simulink model "Validation_Observer"  (R2025b)
settings: Solver=ode15s  StartTime=0.0  StopTime=6  RelTol=1e-3
undefined symbols (not defined in the file): A11, A12, A21, A22, Bd1, Bd2, Bu1, Bu2, CA_re, CAin_re, CB_re, L, QH_re, Qin_V_re, T_re, Tc_re, Tin_re
settings Model: Creator=Lenovo  LastModifiedBy=Lenovo

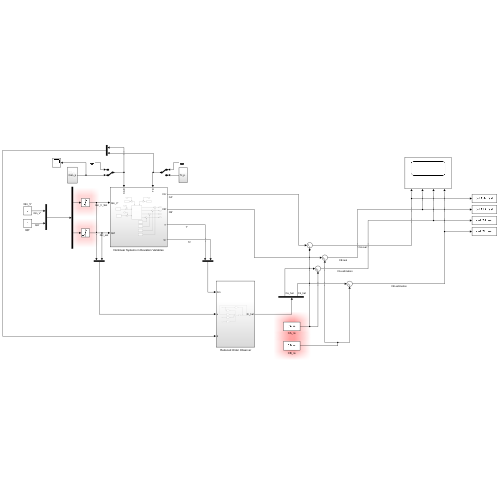
[thumbnail: Simulink's stored preview of the top-level diagram]
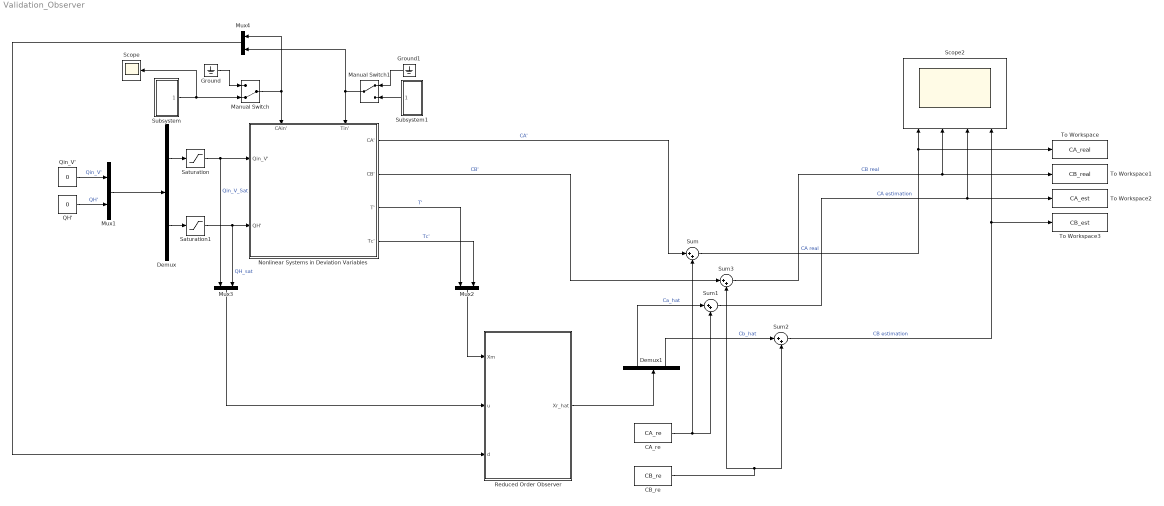
== system Validation_Observer ==
  " Reduced Order Observer" : Subsystem
  CA_re : Constant  Value=CA_re
  CB_re : Constant  Value=CB_re
  Demux : Demux  Outputs=2
  Demux1 : Demux  Outputs=2
  Ground : Ground
  Ground1 : Ground
  Manual Switch : ManualSwitch  CurrentSetting=0
  Manual Switch1 : ManualSwitch
  Mux{1..4} (4 alike) : Mux  Inputs=2
  Nonlinear Systems in Deviation Variables : Subsystem
      settings: PortSchema="{\"entries\":[{\"content\":{\"sides\":[{\"content\":{\"connectorIds\":[\"In1\",\"In2\"]},\"type\":\"ConnectorPlacement.EquallySpacedRectSide\",\"uuid\":\"3cae5363-54ae-4836-a9af-709fc6d72947\"},{\"content\":{\"connectorIds\":[\"Out1\",\"Out2\",\"Out3\",\"Out4\"],\"side\":\"RIGHT\"},\"type\":\"ConnectorPlacement.EquallySpacedRectSide\",\"uuid\":\"ac34fbf0-7c91-43b5-9805-8d79849dc8bb\"},{\"content\":{\"connectorIds\":[\"In3\",\"In4\"],\"side\":\"TOP\"},\"type\":\"ConnectorPlacement.EquallySpacedRectSide\",\"uuid\":\"0c613297-952e-4fe2-85b3-8b705fa3960d\"}]},\"type\":\"ConnectorPlacement.EquallySpacedConnector\",\"uuid\":\"6a9d9fd9-ed65-4660-8ac2-43953dadb3cb\"}],\"packageUris\":[\"http://schema.mathworks.com/mf0/Connector/R2020b\"],\"version\":\"1.0\"}"
  QH' : Constant  Value=0
  Qin_V' : Constant  Value=0
  Saturation : Saturate  UpperLimit=35-Qin_V_re  LowerLimit=5-Qin_V_re
  Saturation1 : Saturate  UpperLimit=0-QH_re  LowerLimit=-8500-QH_re
  Scope : Scope
      settings: ActiveDisplayYMinimum=-1  ActiveDisplayYMaximum=1
  Scope2 : Scope  NumInputPorts=4
      settings: ActiveDisplayYMinimum=-149.80536396754488  ActiveDisplayYMaximum=256.89603505828842  DataLoggingVariableName=ScopeData2
  Subsystem : Subsystem
  Subsystem1 : Subsystem
  Sum{,1..3} (4 alike) : Sum  Inputs=|++
  To Workspace : ToWorkspace  VariableName=CA_real  SaveFormat=Structure With Time  SampleTime=-1
  To Workspace1 : ToWorkspace  VariableName=CB_real  SaveFormat=Structure With Time  SampleTime=-1
  To Workspace2 : ToWorkspace  VariableName=CA_est  SaveFormat=Structure With Time  SampleTime=-1
  To Workspace3 : ToWorkspace  VariableName=CB_est  SaveFormat=Structure With Time  SampleTime=-1
  wires:
  Nonlinear Systems in Deviation Variables/4(Tc') -> Mux2/2  "Tc'"
  Demux/1 -> Saturation/1
  Subsystem/1(Cain_p) -> Scope/1, Manual Switch/2
  Manual Switch/1 -> Nonlinear Systems in Deviation Variables/3(CAin'), Mux4/1
  Qin_V'/1 -> Mux1/1  "Qin_V'"
  Demux/2 -> Saturation1/1
  Ground/1 -> Manual Switch/1
  Mux4/1 -> " Reduced Order Observer"/3(d)
  Mux2/1 -> " Reduced Order Observer"/1(Xm)
  Subsystem1/1(Tc_p) -> Manual Switch1/2
  Manual Switch1/1 -> Mux4/2, Nonlinear Systems in Deviation Variables/4(Tin')
  QH'/1 -> Mux1/2  "QH'"
  Nonlinear Systems in Deviation Variables/3(T') -> Mux2/1  "T'"
  Mux3/1 -> " Reduced Order Observer"/2(u)
  Saturation/1 -> Mux3/1, Nonlinear Systems in Deviation Variables/1(Qin_V')  "Qin_V_Sat"
  Saturation1/1 -> Nonlinear Systems in Deviation Variables/2(QH'), Mux3/2  "QH_sat"
  Ground1/1 -> Manual Switch1/1
  " Reduced Order Observer"/1(Xr_hat) -> Demux1/1
  Mux1/1 -> Demux/1
  Sum/1 -> To Workspace/1, Scope2/1  "CA real"
  Sum1/1 -> To Workspace2/1, Scope2/3  "CA estimation"
  Demux1/1 -> Sum1/1  "Ca_hat"
  Nonlinear Systems in Deviation Variables/1(CA') -> Sum/1  "CA'"
  CA_re/1 -> Sum1/2, Sum/2
  Sum2/1 -> To Workspace3/1, Scope2/4  "CB estimation"
  Demux1/2 -> Sum2/1  "Cb_hat"
  CB_re/1 -> Sum2/2, Sum3/2
  Sum3/1 -> To Workspace1/1, Scope2/2  "CB real"
  Nonlinear Systems in Deviation Variables/2(CB') -> Sum3/1  "CB'"

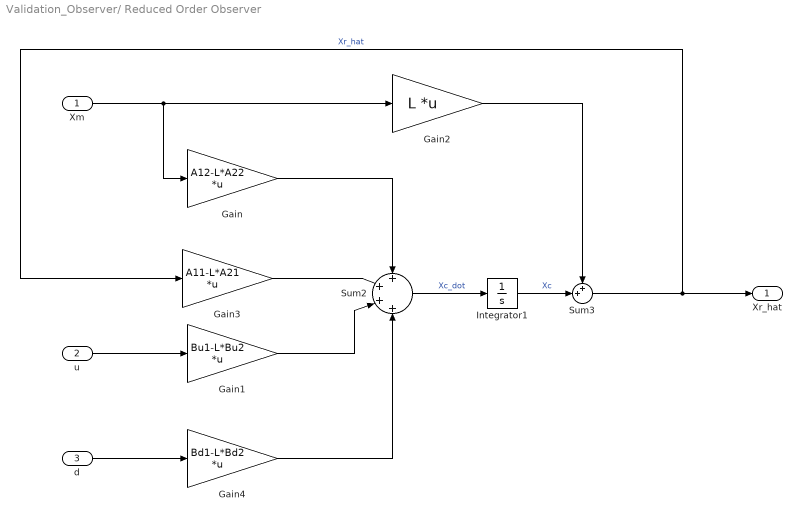
== system Validation_Observer/ Reduced Order Observer ==
  Xm : Inport
  u : Inport  Port=2
  d : Inport  Port=3
  Gain : Gain  Gain=A12-L*A22  Multiplication=Matrix(K*u)
  Gain1 : Gain  Gain=Bu1-L*Bu2  Multiplication=Matrix(K*u)
  Gain2 : Gain  Gain=L  Multiplication=Matrix(K*u)
  Gain3 : Gain  Gain=A11-L*A21  Multiplication=Matrix(K*u)
  Gain4 : Gain  Gain=Bd1-L*Bd2  Multiplication=Matrix(K*u)
  Integrator1 : Integrator
  Sum2 : Sum  Inputs=+|+|+|+
  Sum3 : Sum  Inputs=++|
  Xr_hat : Outport
  wires:
  Gain1/1 -> Sum2/3
  Sum3/1 -> Gain3/1, Xr_hat/1  "Xr_hat"
  Xm/1 -> Gain/1, Gain2/1
  Integrator1/1 -> Sum3/2  "Xc"
  Gain2/1 -> Sum3/1
  Gain/1 -> Sum2/1
  Gain3/1 -> Sum2/2
  Sum2/1 -> Integrator1/1  "Xc_dot"
  u/1 -> Gain1/1
  Gain4/1 -> Sum2/4
  d/1 -> Gain4/1

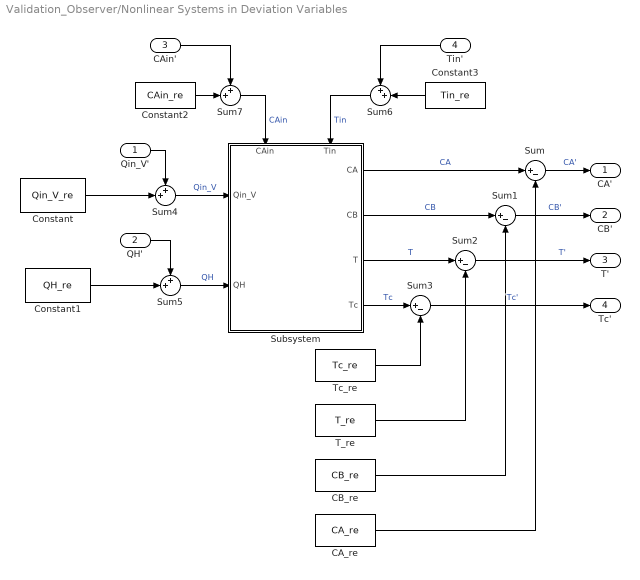
== system Validation_Observer/Nonlinear Systems in Deviation Variables ==
  Qin_V' : Inport
  QH' : Inport  Port=2
  CAin' : Inport  Port=3
  Tin' : Inport  Port=4
  CA_re : Constant  Value=CA_re
  CB_re : Constant  Value=CB_re
  Constant : Constant  Value=Qin_V_re
  Constant1 : Constant  Value=QH_re
  Constant2 : Constant  Value=CAin_re
  Constant3 : Constant  Value=Tin_re
  Subsystem : Subsystem
      settings: PortSchema="{\"entries\":[{\"content\":{\"sides\":[{\"content\":{\"connectorIds\":[\"In1\",\"In2\"]},\"type\":\"ConnectorPlacement.EquallySpacedRectSide\",\"uuid\":\"3cae5363-54ae-4836-a9af-709fc6d72947\"},{\"content\":{\"connectorIds\":[\"Out1\",\"Out2\",\"Out3\",\"Out4\"],\"side\":\"RIGHT\"},\"type\":\"ConnectorPlacement.EquallySpacedRectSide\",\"uuid\":\"ac34fbf0-7c91-43b5-9805-8d79849dc8bb\"},{\"content\":{\"connectorIds\":[\"In3\",\"In4\"],\"side\":\"TOP\"},\"type\":\"ConnectorPlacement.EquallySpacedRectSide\",\"uuid\":\"0c613297-952e-4fe2-85b3-8b705fa3960d\"}]},\"type\":\"ConnectorPlacement.EquallySpacedConnector\",\"uuid\":\"6a9d9fd9-ed65-4660-8ac2-43953dadb3cb\"}],\"packageUris\":[\"http://schema.mathworks.com/mf0/Connector/R2020b\"],\"version\":\"1.0\"}"
  Sum{,1..3} (4 alike) : Sum  Inputs=|+-
  Sum{4..7} (4 alike) : Sum  Inputs=++|
  T_re : Constant  Value=T_re
  Tc_re : Constant  Value=Tc_re
  CA' : Outport
  CB' : Outport  Port=2
  T' : Outport  Port=3
  Tc' : Outport  Port=4
  wires:
  Tc_re/1 -> Sum3/2
  Subsystem/4(Tc) -> Sum3/1  "Tc"
  Subsystem/3(T) -> Sum2/1  "T"
  Sum1/1 -> CB'/1  "CB'"
  Sum4/1 -> Subsystem/1(Qin_V)  "Qin_V"
  CB_re/1 -> Sum1/2
  Sum2/1 -> T'/1  "T'"
  Subsystem/1(CA) -> Sum/1  "CA"
  Sum/1 -> CA'/1  "CA'"
  Constant/1 -> Sum4/2
  T_re/1 -> Sum2/2
  Sum5/1 -> Subsystem/2(QH)  "QH"
  Constant1/1 -> Sum5/2
  CA_re/1 -> Sum/2
  Subsystem/2(CB) -> Sum1/1  "CB"
  QH'/1 -> Sum5/1
  Sum3/1 -> Tc'/1  "Tc'"
  Qin_V'/1 -> Sum4/1
  Constant3/1 -> Sum6/2
  Sum6/1 -> Subsystem/4(Tin)  "Tin"
  Tin'/1 -> Sum6/1
  Sum7/1 -> Subsystem/3(CAin)  "CAin"
  Constant2/1 -> Sum7/2
  CAin'/1 -> Sum7/1

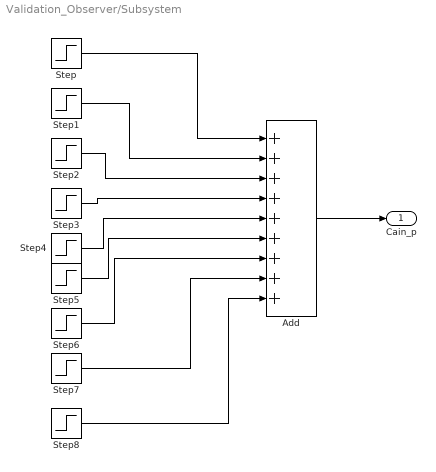
== system Validation_Observer/Subsystem ==
  Add : Sum  Inputs=+++++++++
  Step : Step  Time=0.5  After=300  SampleTime=0
  Step1 : Step  Before=300  After=150  SampleTime=0
  Step2 : Step  Time=1.5  After=-100*2  SampleTime=0
  Step3 : Step  Time=2  Before=-100*2  After=0  SampleTime=0
  Step4 : Step  Time=3  After=100  SampleTime=0
  Step5 : Step  Time=3.5  Before=100  After=50  SampleTime=0
  Step6 : Step  Time=4  Before=300  After=-100  SampleTime=0
  Step7 : Step  Time=4.5  Before=-100  After=130  SampleTime=0
  Step8 : Step  Time=5  Before=130  After=0  SampleTime=0
  Cain_p : Outport
  wires:
  Step/1 -> Add/1
  Step1/1 -> Add/2
  Step2/1 -> Add/3
  Step3/1 -> Add/4
  Add/1 -> Cain_p/1
  Step4/1 -> Add/5
  Step5/1 -> Add/6
  Step6/1 -> Add/7
  Step7/1 -> Add/8
  Step8/1 -> Add/9

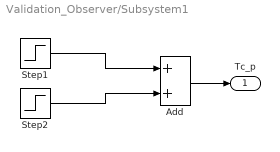
== system Validation_Observer/Subsystem1 ==
  Add : Sum
  Step1 : Step  After=10*2  SampleTime=0
  Step2 : Step  Time=2  Before=10  After=0  SampleTime=0
  Tc_p : Outport
  wires:
  Add/1 -> Tc_p/1
  Step1/1 -> Add/1
  Step2/1 -> Add/2

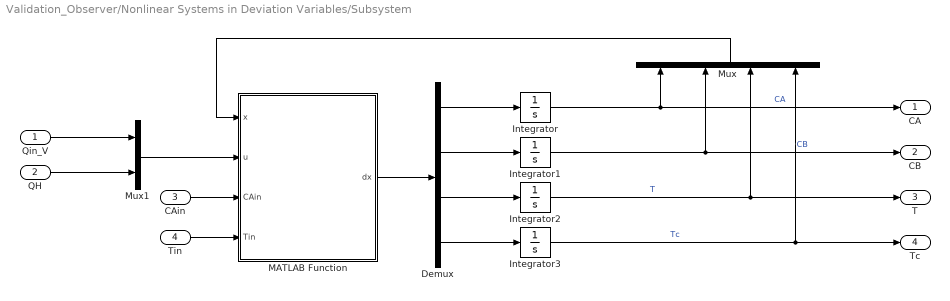
== system Validation_Observer/Nonlinear Systems in Deviation Variables/Subsystem ==
  Qin_V : Inport
  QH : Inport  Port=2
  CAin : Inport  Port=3
  Tin : Inport  Port=4
  Demux : Demux
  Integrator : Integrator  InitialCondition=CA_re
  Integrator1 : Integrator  InitialCondition=CB_re
  Integrator2 : Integrator  InitialCondition=T_re
  Integrator3 : Integrator  InitialCondition=Tc_re
  MATLAB Function : MATLAB Function  TreatAsAtomicUnit=on
  Mux : Mux
  Mux1 : Mux  Inputs=2
  CA : Outport
  CB : Outport  Port=2
  T : Outport  Port=3
  Tc : Outport  Port=4
  wires:
  Demux/3 -> Integrator2/1
  Integrator1/1 -> CB/1, Mux/2  "CB"
  Integrator/1 -> CA/1, Mux/1  "CA"
  Mux/1 -> MATLAB Function/1(x)
  Integrator2/1 -> T/1, Mux/3  "T"
  Integrator3/1 -> Tc/1, Mux/4  "Tc"
  MATLAB Function/1(dx) -> Demux/1
  Demux/2 -> Integrator1/1
  Demux/4 -> Integrator3/1
  Demux/1 -> Integrator/1
  Mux1/1 -> MATLAB Function/2(u)
  Tin/1 -> MATLAB Function/4(Tin)
  QH/1 -> Mux1/2
  CAin/1 -> MATLAB Function/3(CAin)
  Qin_V/1 -> Mux1/1

== matlab function Validation_Observer/Nonlinear Systems in Deviation Variables/Subsystem/MATLAB Function ==
  data: x input; u input; dx output; CAin input; Tin input
function dx = cstr_model(x, u, CAin, Tin)
dx = [0; 0; 0; 0]; 

% State variables

CA = x(1);
CB = x(2);
T  = x(3);
Tc = x(4);

% Manipulated variables
Qin_V = u(1);
QH    = u(2);

% Constants

V = 0.01;
Cp = 3.01;
den = 934.2; 
entAB = 4.2;
entBC = -11.0;
entAD = -41.85;
Ar = 0.215;
Kw = 4032;
mK = 5.0;
CpJ = 2.0;
k1_0 = 1.287e12;
k2_0 = 9.043e6;
E1 = -9758.3;
E2 = -8560.0;

% Arrhenius equations 

k1 = k1_0 * exp(E1 / (T + 273.15));
k2 = k2_0 * exp(E2 / (T + 273.15));

% Mass and energy balances

dx(1) = (Qin_V)*(CAin - CA) - k1*CA - k2*CA^2; % dCA/dt

dx(2) = -(Qin_V)*CB + k1*(CA - CB); %dCB/dt

dx(3) = (Qin_V)*(Tin - T) - (1/(den*Cp))*(k1*CA*entAB + k1*CB*entBC + k2*CA^2*entAD) + (Tc - T)*((Ar*Kw)/(den*Cp*V)); %dT/dt

dx(4) = (QH/(mK*CpJ)) + ((Ar*Kw)/(mK*CpJ))*(T - Tc); %dTc/dt

end
